simulink model "SystemSimulation"  (R2026b)
undefined symbols (not defined in the file): enable, measurement, openLoopSetpoint, opmode, reference, slewrate
settings Model: Creator=BenjaminRupp  LastModifiedBy=BenjaminRupp

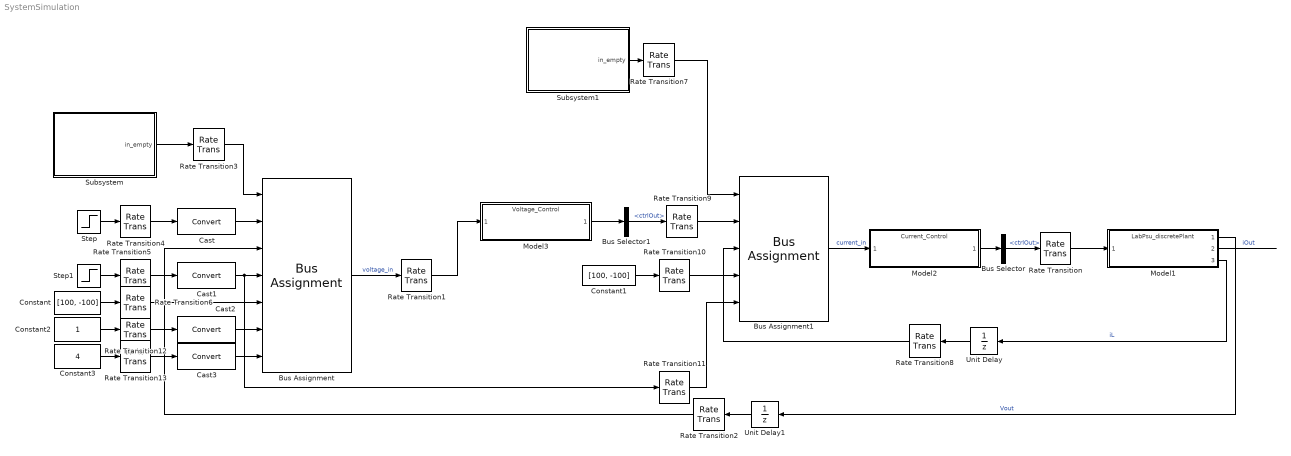
== system SystemSimulation ==
  Bus Assignment : BusAssignment  AssignedSignals=reference,measurement,enable,slewrate,opmode,openLoopSetpoint
  Bus Assignment1 : BusAssignment  AssignedSignals=reference,measurement,slewrate,enable
  Bus Selector : BusSelector  OutputSignals=ctrlOut
  Bus Selector1 : BusSelector  OutputSignals=ctrlOut
  Cast{,1..3} (4 alike) : DataTypeConversion  SaturateOnIntegerOverflow=off  RndMeth=Floor
  Constant : Constant  Value=[100, -100]  OutDataTypeStr=single  SampleTime=-1
  Constant1 : Constant  Value=[100, -100]  OutDataTypeStr=single  SampleTime=-1
  Constant2 : Constant  OutDataTypeStr=single  SampleTime=-1
  Constant3 : Constant  Value=4  OutDataTypeStr=single  SampleTime=-1
  Model1 : ModelReference  ModelNameDialog=LabPsu_discretePlant.slx  SimulationMode=Normal  ModelReferenceVersion=3.0
  Model2 : ModelReference  ModelNameDialog=Current_Control.slx  SimulationMode=Normal  ModelReferenceVersion=3.0
  Model3 : ModelReference  ModelNameDialog=Voltage_Control.slx  SimulationMode=Normal  ModelReferenceVersion=3.0
  Rate Transition : RateTransition
  Rate Transition{1..6,12..13} (8 alike) : RateTransition  OutPortSampleTime=VoltageControl_ts
  Rate Transition{8..11} (4 alike) : RateTransition  OutPortSampleTime=CurrentControl_ts
  Rate Transition7 : RateTransition  OutPortSampleTime=1/10e3
  Step : Step  FinalValue=20  SampleTime=0
  Step1 : Step  SampleTime=0
  Subsystem : Subsystem
  Subsystem1 : Subsystem
  Unit Delay : UnitDelay  SampleTime=-1
  Unit Delay1 : UnitDelay  SampleTime=-1
  wires:
  Model2/1 -> Bus Selector/1
  Bus Selector/1 -> Rate Transition/1  "<ctrlOut>"
  Rate Transition/1 -> Model1/1
  Rate Transition1/1 -> Model3/1
  Subsystem/1(in_empty) -> Rate Transition3/1
  Bus Assignment/1 -> Rate Transition1/1  "voltage_in"
  Model1/1 -> Unit Delay1/1  "Vout"
  Rate Transition2/1 -> Bus Assignment/3
  Rate Transition3/1 -> Bus Assignment/1
  Step/1 -> Rate Transition4/1
  Cast/1 -> Bus Assignment/2
  Rate Transition4/1 -> Cast/1
  Rate Transition5/1 -> Cast1/1
  Step1/1 -> Rate Transition5/1
  Cast1/1 -> Rate Transition11/1, Bus Assignment/4
  Constant/1 -> Rate Transition6/1
  Rate Transition6/1 -> Bus Assignment/5
  Model1/2 -> ?  "iOut"
  Model1/3 -> Unit Delay/1  "iL"
  Model3/1 -> Bus Selector1/1
  Bus Assignment1/1 -> Model2/1  "current_in"
  Subsystem1/1(in_empty) -> Rate Transition7/1
  Rate Transition7/1 -> Bus Assignment1/1
  Constant1/1 -> Rate Transition10/1
  Bus Selector1/1 -> Rate Transition9/1  "<ctrlOut>"
  Rate Transition8/1 -> Bus Assignment1/3
  Rate Transition9/1 -> Bus Assignment1/2
  Rate Transition10/1 -> Bus Assignment1/4
  Rate Transition11/1 -> Bus Assignment1/5
  Unit Delay/1 -> Rate Transition8/1
  Unit Delay1/1 -> Rate Transition2/1
  Cast2/1 -> Bus Assignment/6
  Constant2/1 -> Rate Transition12/1
  Rate Transition12/1 -> Cast2/1
  Rate Transition13/1 -> Cast3/1
  Cast3/1 -> Bus Assignment/7
  Constant3/1 -> Rate Transition13/1

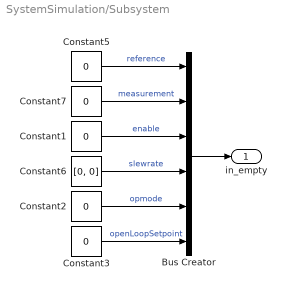
== system SystemSimulation/Subsystem ==
  Bus Creator : BusCreator  Inputs=6  OutDataTypeStr=Bus: VoltageControl_in
  Constant1 : Constant  Value=0  OutDataTypeStr=uint16  SampleTime=-1
  Constant2 : Constant  Value=0  OutDataTypeStr=uint16  SampleTime=-1
  Constant3 : Constant  Value=0  OutDataTypeStr=single  SampleTime=-1
  Constant5 : Constant  Value=0  OutDataTypeStr=single  SampleTime=-1
  Constant6 : Constant  Value=[0, 0]  OutDataTypeStr=single  SampleTime=-1
  Constant7 : Constant  Value=0  OutDataTypeStr=single  SampleTime=-1
  in_empty : Outport
  wires:
  Bus Creator/1 -> in_empty/1
  Constant5/1 -> Bus Creator/1  "reference"
  Constant6/1 -> Bus Creator/4  "slewrate"
  Constant7/1 -> Bus Creator/2  "measurement"
  Constant1/1 -> Bus Creator/3  "enable"
  Constant2/1 -> Bus Creator/5  "opmode"
  Constant3/1 -> Bus Creator/6  "openLoopSetpoint"

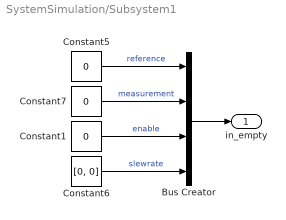
== system SystemSimulation/Subsystem1 ==
  Bus Creator : BusCreator  Inputs=4  OutDataTypeStr=Bus: CurrentControl_in
  Constant1 : Constant  Value=0  OutDataTypeStr=uint16  SampleTime=-1
  Constant5 : Constant  Value=0  OutDataTypeStr=single  SampleTime=-1
  Constant6 : Constant  Value=[0, 0]  OutDataTypeStr=single  SampleTime=-1
  Constant7 : Constant  Value=0  OutDataTypeStr=single  SampleTime=-1
  in_empty : Outport
  wires:
  Constant1/1 -> Bus Creator/3  "enable"
  Constant7/1 -> Bus Creator/2  "measurement"
  Constant6/1 -> Bus Creator/4  "slewrate"
  Constant5/1 -> Bus Creator/1  "reference"
  Bus Creator/1 -> in_empty/1
